simulink model "hunt&hunter"  (R2021b)
settings: Solver=VariableStepAuto  StartTime=0.0  StopTime=50  RelTol=1e-3
settings Model: Creator=kourosh  LastModifiedBy=kourosh

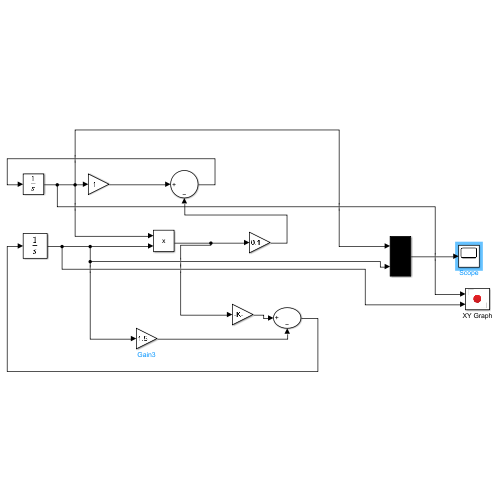
[thumbnail: Simulink's stored preview of the top-level diagram]
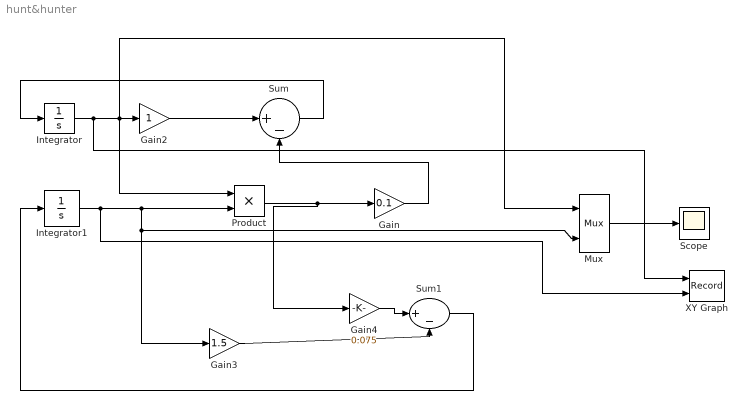
== system hunt&hunter ==
  Gain : Gain  Gain=0.1
  Gain2 : Gain
  Gain3 : Gain  Gain=1.5
  Gain4 : Gain  Gain=0.075
  Integrator : Integrator  InitialCondition=10  ContinuousStateAttributes="\"x\""
  Integrator1 : Integrator  InitialCondition=5
  Mux : Mux  Inputs=2
  Product : Product
  Scope : Scope
  Sum : Sum  Inputs=|+-
  Sum1 : Sum  Inputs=|+-
  XY Graph : Record  FileSettingsInternal="{\"entries\":[{\"content\":{\"excelSettings\":{\"content\":{},\"type\":\"Streamout.ExcelSettings\"}},\"type\":\"Streamout.FileSettingStorage\",\"uuid\":\"149b6535-eb6b-4e87-ba3b-7c4b531b1a96\"}],\"packageUris\":[\"http://schema.mathworks.com/mf0/streamout_blocks/R2020a\"],\"version\":\"1.0\"}"  Layout=[1 1]  SignalsInternal="{\"entries\":[{\"content\":{\"signals\":[{\"content\":{\"blockPath\":[\"untitled/XY Graph\"],\"channel\":[],\"dimensions\":[1],\"domain\":\"untitled/XY Graph\",\"lineColor\":\"#a2142f\",\"plots\":[1],\"port\":1,\"sid\":[\"\"],\"signalID\":236,\"signalName\":\"Integrator\"},\"type\":\"RecordBlkView.Signal\",\"uuid\":\"7d54cf2c-e924-4fbc-9fcf-a71c4c24a223\"},{\"content\":{\"blockPath\":[\"untitled/XY Graph\"],\"channel\":[],\"dimensions\":[1],\"domain\":\"untitled/XY Graph\",\"lineColor\":\"#139fff\",\"plots\":[1],\"port\":2,\"sid\":[\"\"],\"signalID\":240,\"signalName\":\"Integrator1\"},\"type\":\"RecordBlkView.Signal\",\"uuid\":\"6bfc6b71-6ffb-4cbb-a9a7-60335e68222a\"}]},\"type\":\"RecordBlkView.InputSignals\",\"uuid\":\"f96feb8d-c250-4e3f-81ef-3e85a8a6eef0\"}],\"packageUris\":[\"http://schema.mathworks.com/mf0/streamout_blocks/R2020a\"],\"version\":\"1.0\"}"  VisualizationBindings="{\"xyplotplugin\":{\"info\":[{\"series\":[{\"bindingParametersList\":[{\"parameter\":\"X-Axis\",\"signalID\":236,\"signalName\":\"Integrator\"},{\"parameter\":\"Y-Axis\",\"signalID\":240,\"signalName\":\"Integrator1\"}],\"seriesID\":44328}],\"subplotID\":1}]}}"  CompatibilityTag=XY
  wires:
  Integrator/1 -> XY Graph/1, Product/1, Mux/1, Gain2/1
  Integrator1/1 -> XY Graph/2, Gain3/1, Mux/2, Product/2
  Gain2/1 -> Sum/1
  Product/1 -> Gain4/1, Gain/1
  Gain/1 -> Sum/2
  Sum/1 -> Integrator/1
  Gain3/1 -> Sum1/2
  Sum1/1 -> Integrator1/1
  Mux/1 -> Scope/1
  Gain4/1 -> Sum1/1
